simulink model "turbo_controller"  (R2025a)
settings: Solver=FixedStepAuto  StartTime=0.0  StopTime=inf  FixedStep=0.001  RelTol=1e-3
PostLoadFcn:
  | % 自动定位同目录CubeMX文件；不需要外部初始化脚本。
  | codertarget.data.setParameterValue('turbo_controller','STM32CubeMX.ProjectFile',fullfile(fileparts(get_param('turbo_controller','FileName')),'turbo_f407.ioc'));
InitFcn:
  | % 中文说明：按原控制器字段与类型创建三组接口总线；控制参数已内嵌。
  | tc_names=["EValve_Cycle" "EValve_Open" "Eblast_Cycle" "Eblast_Open" "Motor_Cycle" "Motor_Open" "EValve_Enable" "Eblast_Enable" "Motor_Enable" "SWO_Firework" "SWO_BleedAir" "EngineState" "Flag_ECUReset_Clear" "Flag_ECUReset_Save" "Flag_Reset_Enable" "Accelerator" "Nc_dem" "Nc"]; tc_types=["uint16" "uint16" "uint16" "uint16" "uint16" "uint16" "uint8" "uint8" "uint8" "uint8" "uint8" "uint8" "uint8" "uint8" "uint8" "single" "single" "single"];
  | for tc_k=1:numel(tc_names)
  |  tc_e(tc_k)=Simulink.BusElement; tc_e(tc_k).Name=char(tc_names(tc_k)); tc_e(tc_k).DataType=char(tc_types(tc_k));
  | end
  | EngineControl_Out=Simulink.Bus; EngineControl_Out.DataScope='Exported'; EngineControl_Out.Elements=tc_e;
  | clear tc_e tc_names tc_types tc_k
  | tc_names=["savedata1" "savedata2" "savedata3" "savedata4" "savedata5" "savedata6" "savedata7" "savedata8" "savedata9" "savedata10" "savedata11" "savedata12" "savedata13" "savedata14" "savedata15" "savedata16" "savedata17" "savedata18" "savedata19" "savedata20" "savedata21" "savedata22" "savedata23" "savedata24" "savedata25"]; tc_types=["single" "single" "single" "single" "single" "single" "single" "single" "single" "single" "single" "single" "single" "single" "single" "single" "single" "single" "single" "single" "single" "single" "single" "single" "single"];
  | for tc_k=1:numel(tc_names)
  |  tc_e(tc_k)=Simulink.BusElement; tc_e(tc_k).Name=char(tc_names(tc_k)); tc_e(tc_k).DataType=char(tc_types(tc_k));
  | end
  | SaveData_Out=Simulink.Bus; SaveData_Out.DataScope='Exported'; SaveData_Out.Elements=tc_e;
  | clear tc_e tc_names tc_types tc_k
  | tc_names=["senddata1" "senddata2" "senddata3" "senddata4" "senddata5" "senddata6" "senddata7" "senddata8" "senddata9" "senddata10" "senddata11" "senddata12" "senddata13" "senddata14" "senddata15" "senddata16" "senddata17" "senddata18" "senddata19" "senddata20" "senddata21" "senddata22" "senddata23" "senddata24" "senddata25" "senddata26" "senddata27" "senddata28" "senddata29"]; tc_types=["uint8" "uint8" "uint8" "uint8" "uint8" "uint8" "uint8" "uint8" "uint8" "uint8" "uint8" "uint8" "uint8" "uint8" "uint8" "uint8" "uint8" "uint8" "uint8" "uint8" "uint8" "uint8" "uint8" "uint8" "uint8" "uint8" "uint8" "uint8" "uint8"];
  | for tc_k=1:numel(tc_names)
  |  tc_e(tc_k)=Simulink.BusElement; tc_e(tc_k).Name=char(tc_names(tc_k)); tc_e(tc_k).DataType=char(tc_types(tc_k));
  | end
  | SendData_Out=Simulink.Bus; SendData_Out.DataScope='Exported'; SendData_Out.Elements=tc_e;
  | clear tc_e tc_names tc_types tc_k
  | 
  | % 以下为接口中文说明；只设置描述，不改变数值或数据类型。
  | EngineControl_Out.Description='执行控制输出（阀、电机、点火、状态及复位请求）';
  | tc_cn=["EValve_Cycle（主油阀周期计数（每计数2毫秒））" "EValve_Open（主油阀开通计数（每计数2毫秒））" "Eblast_Cycle（副油阀周期计数（每计数2毫秒））" "Eblast_Open（副油阀开通计数（每计数2毫秒））" "Motor_Cycle（起动电机周期计数）" "Motor_Open（起动电机开通计数）" "EValve_Enable（主油阀驱动使能）" "Eblast_Enable（副油阀驱动使能）" "Motor_Enable（起动电机使能）" "SWO_Firework（点火器使能（1开））" "SWO_BleedAir（引气阀使能（1开））" "EngineState（发动机状态）" "Flag_ECUReset_Clear（清除复位恢复状态请求）" "Flag_ECUReset_Save（保存复位恢复数据请求）" "Flag_Reset_Enable（处理器软件复位请求）" "Accelerator（油门／油泵给定控制量）" "Nc_dem（控制目标转速）" "Nc（发动机反馈转速（转每分））"];
  | tc_elements=EngineControl_Out.Elements;
  | for tc_k=1:numel(tc_cn)
  |  tc_elements(tc_k).Description=char(tc_cn(tc_k));
  | end
  | EngineControl_Out.Elements=tc_elements;
  | clear tc_cn tc_elements tc_k
  | SaveData_Out.Description='25项运行记录；字段含义按当前模型数据来源解释';
  | tc_cn=["savedata1（指令回显记录）" "savedata2（入口总温记录（℃））" "savedata3（电源电压记录）" "savedata4（排气温度记录（℃））" "savedata5（标定燃油压力记录）" "savedata6（副油阀占空比记录（％））" "savedata7（主油阀占空比记录（％））" "savedata8（温度修正转速记录）" "savedata9（开关输出及反馈位域）" "savedata10（物理转速记录）" "savedata11（油泵目标给定原始值）" "savedata12（起动电机占空比记录（％））" "savedata13（发动机状态码记录）" "savedata14（故障告警位域记录）" "savedata15（模型记录帧序号）" "savedata16（处理器温度记录（℃））" "savedata17（装订转速记录（沿用旧电源字段名））" "savedata18（导航高度记录）" "savedata19（飞行空速记录）" "savedata20（主阀旧记录位（恒零保留））" "savedata21（第21项保留记录（恒零））" "savedata22（保留记录项22）" "savedata23（保留记录项23）" "savedata24（保留记录项24）" "savedata25（保留记录项25）"];
  | tc_elements=SaveData_Out.Elements;
  | for tc_k=1:numel(tc_cn)
  |  tc_elements(tc_k).Description=char(tc_cn(tc_k));
  | end
  | SaveData_Out.Elements=tc_elements;
  | clear tc_cn tc_elements tc_k
  | SendData_Out.Description='29字段回传及外设命令接口；板端上位机帧只取第3至27字段';
  | tc_cn=["senddata1（回传发送允许标志（不直接上线路））" "senddata2（回传载荷长度25字节）" "senddata3（回传指令回显字节）" "senddata4（总温编码字节（℃＋80））" "senddata5（电源电压编码字节）" "senddata6（排温编码高字节）" "senddata7（排温编码低字节）" "senddata8（燃油压力编码高字节）" "senddata9（燃油压力编码低字节）" "senddata10（副油阀占空比字节（％））" "senddata11（主油阀占空比字节（％））" "senddata12（修正转速编码高字节）" "senddata13（修正转速编码低字节）" "senddata14（驱动及反馈状态位域）" "senddata15（物理转速编码高字节）" "senddata16（物理转速编码低字节）" "senddata17（油泵目标给定高字节（串口二使用））" "senddata18（油泵目标给定低字节（串口二使用））" "senddata19（起动电机占空比命令（串口一使用））" "senddata20（发动机状态码字节）" "senddata21（故障告警位域字节）" "senddata22（帧序号占位（板端另行填写））" "senddata23（处理器温度编码（℃＋50））" "senddata24（控制目标转速编码高字节）" "senddata25（控制目标转速编码低字节）" "senddata26（占位字节（板端改填实测泵速高字节））" "senddata27（占位字节（板端改填实测泵速低字节））" "senddata28（装订转速高字节（本板未发送））" "senddata29（装订转速低字节（本板未发送））"];
  | tc_elements=SendData_Out.Elements;
  | for tc_k=1:numel(tc_cn)
  |  tc_elements(tc_k).Description=char(tc_cn(tc_k));
  | end
  | SendData_Out.Elements=tc_elements;
  | clear tc_cn tc_elements tc_k
  | 
  | 
  | % FRAM模块化事务：接口类型和上电初始状态，随模型保存，无外部初始化文件。
  | clear FM_elements
  | FM_elements(1)=Simulink.BusElement;FM_elements(1).Name='phase';FM_elements(1).DataType='uint8';FM_elements(1).Dimensions=[1 1];FM_elements(1).Description='phase（当前事务阶段）';
  | FM_elements(2)=Simulink.BusElement;FM_elements(2).Name='a';FM_elements(2).DataType='uint8';FM_elements(2).Dimensions=[64 1];FM_elements(2).Description='a（启动时缓存的首区64字节）';
  | FM_elements(3)=Simulink.BusElement;FM_elements(3).Name='active';FM_elements(3).DataType='uint16';FM_elements(3).Dimensions=[1 1];FM_elements(3).Description='active（当前有效记录区地址）';
  | FM_elements(4)=Simulink.BusElement;FM_elements(4).Name='generation';FM_elements(4).DataType='uint32';FM_elements(4).Dimensions=[1 1];FM_elements(4).Description='generation（当前有效记录代号）';
  | FM_elements(5)=Simulink.BusElement;FM_elements(5).Name='record';FM_elements(5).DataType='uint8';FM_elements(5).Dimensions=[64 1];FM_elements(5).Description='record（本次冻结的待写记录）';
  | FM_elements(6)=Simulink.BusElement;FM_elements(6).Name='addr';FM_elements(6).DataType='uint16';FM_elements(6).Dimensions=[1 1];FM_elements(6).Description='addr（本次备用写入地址）';
  | FM_elements(7)=Simulink.BusElement;FM_elements(7).Name='lastSave';FM_elements(7).DataType='single';FM_elements(7).Dimensions=[1 1];FM_elements(7).Description='lastSave（上次开始保存的秒数）';
  | FM_elements(8)=Simulink.BusElement;FM_elements(8).Name='lastState';FM_elements(8).DataType='uint8';FM_elements(8).Dimensions=[1 1];FM_elements(8).Description='lastState（上次保存时的发动机状态）';
  | FM_elements(9)=Simulink.BusElement;FM_elements(9).Name='boot';FM_elements(9).DataType='boolean';FM_elements(9).Dimensions=[1 1];FM_elements(9).Description='boot（启动记录是否允许恢复）';
  | FM_elements(10)=Simulink.BusElement;FM_elements(10).Name='consumed';FM_elements(10).DataType='boolean';FM_elements(10).Dimensions=[1 1];FM_elements(10).Description='consumed（本次启动恢复通知是否已发送）';
  | FM_elements(11)=Simulink.BusElement;FM_elements(11).Name='payload';FM_elements(11).DataType='uint8';FM_elements(11).Dimensions=[20 1];FM_elements(11).Description='payload（当前20字节恢复内容）';
  | ... (+35 lines)
model workspace (MAT data in the model file):
  CRC16_Table_Reference = [0 4129 8258 12387 16516 20645 24774 28903 33032 37161 41290 45419 ... (256 elements, 256x1)]
  PE_Kaer = [0.15402 0.15402 0.12264 0.10076 0.09481 0.07601 0.07111 0.0569 0.05198 0.04926 0.05308 0.04325 ... (13 elements, 1x13)]
  PE_Nr = [21.2982 61.4260372 67.7475458 72.7394382 76.845934 80.6988798 83.8449282 86.6491912 88.9382406 89.178606 91.1938214 93.4068058 ... (13 elements, 1x13)]
  PE_Pump_Translate = 33.5999984741
  PE_RotaSpeed_Translate = 860
  PE_Taer = [0.4939154 0.4939154 0.40780982 0.34066978 0.31622756 0.30405716 0.34300244 0.26785022 0.37393554 0.23914836 0.44563948 0.31044662 ... (13 elements, 1x13)]
  PF_ACCFULLRANGE = 3360
  PF_Flag_ECUReset = 0
  PF_Flag_rx_suc = 1
  PF_Gear_Info = [40000; 45000; 50000; 55000; 57000; 59000; 60000; 61000; 61000; 61000; 61000; 61000]
  PF_K_TiaoJie = 1
  PF_Kpu = 10
  PF_MySet_Rxdata = [0 0 0 0 0 0 0 0 0 0 0 0 ... (50 elements, 50x1)]
  PF_MyUsart1_Rxdata = [0 0 0 0 0 0 0 0 0 0 0 0 ... (50 elements, 50x1)]
  PF_MyUsart2_Rxdata = [0 0 0 0 0 0 0 0 0 0 0 0 ... (50 elements, 50x1)]
  PF_Reset_Information = [0 0 0 0 0 0 0 0 0 0 0 0 ... (20 elements, 20x1)]
  PF_Sensor_X1_T4 = [0 4095]
  PF_Sensor_X2_T4 = [0 1.66666698456]
  PF_Sensor_X3_T4 = [0 504 999 1497 2010 2529 3051 3568 4076 4571 4959]
  PF_Sensor_X_P2 = [0.5 3]
  PF_Sensor_X_Poil = [0.5 3]
  PF_Sensor_X_T1t = [-50 300]
  PF_Sensor_X_Vpower = [0 3]
  PF_Sensor_X_Vpump = [0 3]
  PF_Sensor_Y1_T4 = [0 3]
  PF_Sensor_Y2_T4 = [0 5000]
  PF_Sensor_Y3_T4 = [0 100 200 300 400 500 600 700 800 900 980]
  PF_Sensor_Y_P2 = [0 1000]
  PF_Sensor_Y_Poil = [0 1000]
  PF_Sensor_Y_T1t = [-50 300]
  PF_Sensor_Y_Vpower = [0 33]
  PF_Sensor_Y_Vpump = [0 33]
  PG_CtrlMode_CloseLoop : mpt.Parameter (value not decoded)
  PG_CtrlMode_ManualAcc : mpt.Parameter (value not decoded)
  PG_CtrlMode_Origin : mpt.Parameter (value not decoded)
  PG_CtrlMode_Start : mpt.Parameter (value not decoded)
  PG_CtrlMode_Stop : mpt.Parameter (value not decoded)
  PG_ES_Clp : mpt.Parameter (value not decoded)
  PG_ES_EngStart : mpt.Parameter (value not decoded)
  PG_ES_Manual : mpt.Parameter (value not decoded)
  PG_ES_Origin : mpt.Parameter (value not decoded)
  PG_ES_Stop : mpt.Parameter (value not decoded)
  PG_Instr_BleedAirSet : mpt.Parameter (value not decoded)
  PG_Instr_CloseLoop : mpt.Parameter (value not decoded)
  PG_Instr_ECUReSet : mpt.Parameter (value not decoded)
  PG_Instr_EValveSet : mpt.Parameter (value not decoded)
  PG_Instr_EblastSet : mpt.Parameter (value not decoded)
  PG_Instr_Erase : mpt.Parameter (value not decoded)
  PG_Instr_FireWorkSet : mpt.Parameter (value not decoded)
  PG_Instr_ManualPlus : mpt.Parameter (value not decoded)
  PG_Instr_ManualrReduce : mpt.Parameter (value not decoded)
  PG_Instr_MotorSet : mpt.Parameter (value not decoded)
  PG_Instr_OilSet : mpt.Parameter (value not decoded)
  PG_Instr_SelfCheck : mpt.Parameter (value not decoded)
  PG_Instr_Start : mpt.Parameter (value not decoded)
  PG_Instr_Stop : mpt.Parameter (value not decoded)
  PG_Instr_StopZero : Simulink.Parameter (value not decoded)
  PG_Location_Air : Simulink.Parameter (value not decoded)
  PG_Location_Gnd : Simulink.Parameter (value not decoded)
  PG_ServoCtrlMode_CloseLoop : Simulink.Parameter (value not decoded)
  PG_ServoCtrlMode_CloseLoopMax : Simulink.Parameter (value not decoded)
  PG_ServoCtrlMode_CloseLoopMin : Simulink.Parameter (value not decoded)
  PG_ServoCtrlMode_ManualAcc : Simulink.Parameter (value not decoded)
  PG_ServoCtrlMode_ManualAccMax : Simulink.Parameter (value not decoded)
  PG_ServoCtrlMode_ManualAccMin : Simulink.Parameter (value not decoded)
  PG_SpeedDot_Permit : Simulink.Parameter (value not decoded)
  PL_EngineModel_Actuator = [0 10 100]
  PL_EngineModel_EngineStar_Press_P2 = [1013 1098.4 1099.144828 1099.931034 1103.613793 1162.662069 1143.793103 1131.006897 1123.186207 1117.6 1114 1111.806897 ... (127 elements, 1x127)]
  PL_EngineModel_EngineStar_RotaSpeed = [200 2000 9584 9660 10220 10240 10260 10288 10308 10368 10380 10408 ... (127 elements, 1x127)]
  PL_EngineModel_EngineStar_Temp_Exhaust = [128 129 129.1 130 131 131.1 132 133 134 134.1 135 135.1 ... (127 elements, 1x127)]
  PL_EngineModel_EngineStar_Time = [0.05 0.1 0.15 0.2 0.25 0.3 0.35 0.4 0.45 0.5 0.55 0.6 ... (127 elements, 1x127)]
  PL_EngineModel_IdleAbove_Nr = [0 21.2982 61.4260372 67.7475458 72.7394382 76.845934 80.6988798 83.8449282 86.6491912 88.9382406 89.178606 91.1938214 ... (14 elements, 1x14)]
  PL_EngineModel_IdleAbove_P2r = [0.986923266716 1.57907722675 1.81593881076 1.99358499877 2.23044658278 2.43770046879 2.65482358747 2.84233900814 3.03972366149 3.18776215149 3.25684678016 3.3950160375 ... (14 elements, 1x14)]
  PL_EngineModel_IdleAbove_Tempr = [0.0536001429337 1.07200285867 1.63301768805 1.63659103091 1.66875111667 1.72592460247 1.77595140254 1.86171163123 1.95461854565 2.03323208862 2.03323208862 2.13685903162 ... (14 elements, 1x14)]
  PL_EngineModel_IdleAbove_Ter = [0.42434128 0.42434128 0.42434128 0.30669408 0.23570008 0.22150128 0.1997974 0.23803274 0.16115638 0.24279948 0.13600422 0.31308354 ... (14 elements, 1x14)]
  PL_EngineModel_IdleAbove_Wfr = [0 10.142 23.8337 27.8905 31.9473 36.0041 40.0609 44.1177 48.1745 52.2313 52.7384 56.7952 ... (14 elements, 1x14)]
  PL_EngineModel_Press_P2 = [400 400 400 400 400 400 400 400 400 400]
  PL_EngineModel_Rotaspeed = [0 20000 96400]
  PL_EngineModel_Temp_Exhaust = [500 500 500 500 500 500 500 500 500 500]
  PL_Kaer = [0.1 0.1 0.1 0.1 0.1 0.1]
  PL_Nr = [50 60 70 80 90 100]
  PL_Taer = [0.1 0.1 0.1 0.1 0.1 0.1]
  Sig : Simulink.Signal (value not decoded)
  Ts_ms : Simulink.Parameter (value not decoded)
  false : Simulink.Parameter (value not decoded)
  true : Simulink.Parameter (value not decoded)
symbols that are objects in the model workspace (value not decoded): PG_CtrlMode_CloseLoop, PG_CtrlMode_ManualAcc, PG_CtrlMode_Origin, PG_CtrlMode_Start, PG_CtrlMode_Stop, PG_ES_Clp, PG_ES_EngStart, PG_ES_Manual, PG_ES_Origin, PG_ES_Stop, PG_Instr_BleedAirSet, PG_Instr_CloseLoop, PG_Instr_EblastSet, PG_Instr_ECUReSet, PG_Instr_Erase, PG_Instr_EValveSet, PG_Instr_FireWorkSet, PG_Instr_ManualPlus, PG_Instr_ManualrReduce, PG_Instr_MotorSet, PG_Instr_OilSet, PG_Instr_SelfCheck, PG_Instr_Start, PG_Instr_Stop, PG_Instr_StopZero, PG_ServoCtrlMode_CloseLoop, PG_ServoCtrlMode_CloseLoopMax, PG_ServoCtrlMode_CloseLoopMin, PG_ServoCtrlMode_ManualAcc, PG_ServoCtrlMode_ManualAccMax, PG_ServoCtrlMode_ManualAccMin, Ts_ms
libraries: simulink x97, stm32blockslib x10, stm32f4xxblockslib x8
(part 5 of 26)

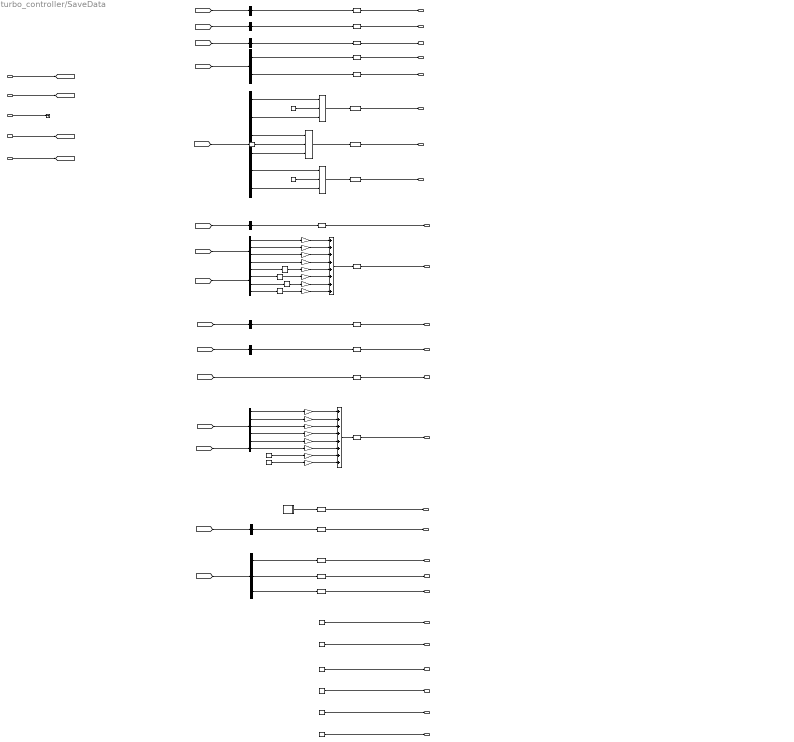
== system turbo_controller/SaveData ==
  note: SaveData的职责：整理25项运行记录，不直接写文件
      |
      | 从发动机模式、传感器/通信、执行输出和监视告警中取出需要记录的量，按固定25个输出端口排列，
      | 供后面的Savedata总线和LogPack使用。
      |
      | 多数通道只转换为single，不额外加偏置、不拆高低字节。阀门和电机另计算开通比例；开关和告警另
      | 组合为位字段；Hold另产生循环序号。
      |
      | S_ClM_Parameter输入当前直接接Terminator，未参与这些记录。第20～25项目前全部是固定0，不应沿
      | 用旧名称推断这些项已经存了主阀输出、软件版本或其他传感器量。
      |
      | 本页没有文件路径、SD卡写入、SPI写入或串口封帧动作。它提供一组记录字段；实际数据去向还要继
      | 续看LogPack、SDLog和FRAM事务。
  note: 温度、电压、油压和转速：保留数值，不按回传字节编码
      |
      | 第2项T0取Sensor.T0，直接转single，25 ℃仍记录25，不加80。
      | 第3项dianyuandianya取Sensor.Vpower，24 V仍记录24，不乘5。
      | 第4项T4取Sensor.T4_Filter，第5项POil取Sensor.POil_Filter，保留滤波后的值，不拆成两个字节；
      | 油压单位沿用上游标定。
      | 第8项HuanSuanZhuanSu取温度修正转速，第10项WuLiZhuanSu取Sensor.Origin_Nc，保留完整转速，不
      | 除2。
      | 第16项Tecu取Sensor.Tecu，25 ℃仍记录25，不加50。
      | 第11项NBump_MuBiao取执行输出Accelerator，是泵控制给定编码，不是实测泵速。
      |
      | 这些转换的输出类型是single。即使参数页上写有Floor，也不能据此说这里全部取整；浮点转single
      | 不等于转整数，原有小数一般仍保留到single精度。
  note: 阀门和电机记录的是开通比例，不是机械反馈
      |
      | 从S_Servo_Out取Open及Cycle，计算：
      | 第6项副油阀=100×Eblast_Open/Eblast_Cycle；
      | 第7项主油阀=100×EValve_Open/EValve_Cycle；
      | 第12项电机=100×Motor_Open/Motor_Cycle。
      | 结果转single记录，此处没有再转成uint8或强制向下取整。
      |
      | 例周期30、开通15，记录50，代表50%开通比例；周期30、开通10，约为33.3333。它不是开了15 ms，
      | 也不是阀芯走到50%的位置。
      |
      | 这些量来自驱动设定，使能状态另在第9项位字段里。比例非0不自动证明执行器已经动作。本页沿用原
      | 除法，没有在这里增加分母为0时的保护逻辑；本次仅更新说明。
  note: 第9项开关量：命令和取反反馈合成一个数
      |
      | 低四位来自执行输出，高四位来自传感器反馈的逻辑取反：
      | 位0，权重1：SWO_Firework点火使能；
      | 位1，权重2：EValve_Enable主阀使能；
      | 位2，权重4：Eblast_Enable副阀使能；
      | 位3，权重8：SWO_BleedAir引气使能；
      | 位4，权重16：NOT SWI_Firework；
      | 位5，权重32：NOT SWI_EValve；
      | 位6，权重64：NOT SWI_Eblast；
      | 位7，权重128：NOT SWI_BleedAir。
      |
      | 按各位权重相加后转single存储。例只有主阀使能和取反后的主阀反馈为真，记录2+32=34。分析日志
      | 时先转成整数再按位拆解，不要把34当成开度34%。
      |
      | Motor_Enable没有放入这8位；电机开通比例在第12项。高四位与原反馈相反，不能直接当作GPIO原电
      | 平解释。
  note: 第14项告警字段：与SendData的定义存在差别
      |
      | 各布尔量乘位权后相加，结果转single：
      | 位0（1）：Alarm_OverTemp；
      | 位1（2）：Alarm_OverSpeed；
      | 位2（4）：Flag_NcFailure；
      | 位3（8）：Alarm_ECUReset；
      | 位4（16）：Alarm_Vpower_Low；
      | 位5（32）：Sensor.SWI_ValveErr原值；
      | 位6（64）：当前常量0；
      | 位7（128）：当前常量0。
      |
      | 例如超温、欠压为真，其余为假，得到17。这里的位5直接使用SWI_ValveErr，没有NOT；SendData对应
      | 位使用了NOT，不能拿同一套解码说明混用。这里的位6也没有接Lock_NcFailure，记录0不表示该锁存
      | 故障一定不存在。
      |
      | 本页只组合并记录标志，不触发报警、停车或复位。判断运行状态要另外看第13项模式编号。
  note: 25项顺序表：第1～13项
      |
      | 1 ZhiLingHuiChuan：COMM.Instr_XianShi，指令回显。
      | 2 T0：入口温度，直接single。
      | 3 dianyuandianya：Sensor.Vpower，供电电压原值。
      | 4 T4：滤波后排温。
      | 5 POil：滤波后油压。
      | 6 Eblast：副油阀开通比例，100×Open/Cycle。
      | 7 EValve：主油阀开通比例，100×Open/Cycle。
      | 8 HuanSuanZhuanSu：温度修正转速完整值。
      | 9 KaiGuanLiang：命令与取反反馈的8位组合。
      | 10 WuLiZhuanSu：Sensor.Origin_Nc完整值。
      | 11 NBump_MuBiao：Accelerator泵给定控制编码。
      | 12 Motor：电机开通比例，100×Open/Cycle。
      | 13 FaDongJiZhuangTai：EngineState，0初始、1普通起动、2闭环、3手动、4停车。
      |
      | 这些是记录项/输出端口编号，不是串口帧字节位置。第13项是发动机模式，不是指令编号或起动A～F
      | 阶段。
  note: 25项顺序表：第14～25项及旧名称说明
      |
      | 14 GuZhangXingXi：告警位组合，按本页专用位定义解码。
      | 15 zhenjishu：Hold产生的0～255循环序号。
      | 16 Tecu：Sensor.Tecu处理器温度原值，不加50。
      | 17 DianYuan：实际为COMM.SpeedLoad目标/装订转速，不是电源电压。
      | 18 H：COMM.H_Gprs导航高度，沿用输入单位，本页不作单位换算。
      | 19 speed：COMM.AirSpeed飞行空速；不是发动机轴转速。
      | 20 ZhuFaShuChu：当前固定0，不是有效主阀反馈。
      | 21 名称为12：当前固定0，此名字不表示第12项。
      | 22 BeiYong1：固定0。
      | 23 BeiYong2：固定0。
      | 24 BeiYong3：固定0。
      | 25 BeiYong4：固定0。
      |
      | 第17项还会以savedata17被FRAM打包步骤读取，作为恢复记录中的目标转速。若把它误认为电压，会连
      | 带误读恢复信息。真正供电在第3项。
  note: Hold序号与最终27项日志的关系
      |
      | Hold每次执行时判断Out是否达到255：达到则置0，否则加1。序列循环为…253、254、255、0、1…；
      | 第15项把这个序号转single记录。
      |
      | 它是本图执行次数的循环标记，不是时间戳。重复的序号不一定表示重复数据，因为每256次执行就回
      | 到同一编号；不要把序号差直接解释成秒数。
      |
      | 外层LogPack按savedata1～savedata25拼接本页25项，末尾追加第26项时间（秒）和第27项FRAM写后验
      | 证失败次数，形成27×1的single向量。随后SDLog的To Workspace在仿真中生成engine_log。
      |
      | 这里的27项是数值记录，不是27字节帧；名为SDLog也不能单凭名称断言已写入实际SD卡。实际记录周
      | 期取决于外层执行与记录接口，本页没有独立的周期触发器。
  note: 读日志时不要套用SendData的还原规则
      |
      | SaveData与SendData虽然记录同类变量，表示方式不同：
      | 日志T0直接是温度；回传T0加80。
      | 日志Tecu直接是温度；回传Tecu加50且限幅。
      | 日志电压直接是V；回传电压乘5。
      | 日志转速保留完整值；回传部分转速除2并拆字节。
      | 日志主副阀、电机比例是single，可有小数；回传比例转uint8。
      | 日志告警位5是SWI_ValveErr原值，位6为0；回传位5取反，位6接Lock_NcFailure。
      |
      | 例如日志中T0=25、电压=24、转速=50000，应按这些数直接阅读，不能再减80、除5或乘2。开关与告警
      | 则需要按位解析，泵给定仍是控制编码。所有项统一转single不意味着所有项拥有相同单位。
  S_EngineState : Inport
      settings: AttributesFormatString=S_EngineState（发动机状态）
  S_SPM : Inport  Port=2
      settings: AttributesFormatString=S_SPM（通信及传感器信息总线）
  S_ClM_Parameter : Inport  Port=3
      settings: AttributesFormatString=S_ClM_Parameter（控制规律管理模块参数）
  S_Servo_Out : Inport  Port=4
      settings: AttributesFormatString=S_Servo_Out（伺服输出）
  S_MAlarm : Inport  Port=5
      settings: AttributesFormatString=S_MAlarm（报警）
  Bus Selector1 : BusSelector  OutputSignals=Sensor（传感器信息总线）.T0（入口总温）
      settings: AttributesFormatString=Bus Selector1（总线选择器1）
  Bus Selector10 : BusSelector  OutputSignals=EValve_Open（主油阀开通计数）,EValve_Cycle（主油阀周期计数）,Eblast_Open（副油阀开通计数）,Eblast_Cycle（副油阀周期计数）,Motor_Open（起动电机开通计数）,Motor_Cycle（起动电机周期计数）
      settings: AttributesFormatString=Bus Selector10（总线选择器10）
  Bus Selector11 : BusSelector  OutputSignals=SWO_Firework（点火器使能）,EValve_Enable（主油阀使能）,Eblast_Enable（副油阀使能）,SWO_BleedAir（引气阀使能）
      settings: AttributesFormatString=Bus Selector11（总线选择器11）
  Bus Selector12 : BusSelector  OutputSignals=Sensor（传感器信息总线）.Tecu（处理器温度）
      settings: AttributesFormatString=Bus Selector12（总线选择器12）
  Bus Selector13 : BusSelector  OutputSignals=COMM（通信信息总线）.Instr_XianShi（指令回显）
      settings: AttributesFormatString=Bus Selector13（总线选择器13）
  Bus Selector14 : BusSelector  OutputSignals=Sensor（传感器信息总线）.SWI_Firework（点火器告警反馈）,Sensor（传感器信息总线）.SWI_EValve（主油阀反馈）,Sensor（传感器信息总线）.SWI_Eblast（副油阀反馈）,Sensor（传感器信息总线）.SWI_BleedAir（引气阀反馈）
      settings: AttributesFormatString=Bus Selector14（总线选择器14）
  Bus Selector15 : BusSelector  OutputSignals=Accelerator（油泵给定控制量）
      settings: AttributesFormatString=Bus Selector15（总线选择器15）
  Bus Selector17 : BusSelector  OutputSignals=Sensor（传感器信息总线）.HuanSuanZhuanSu（温度修正转速）
      settings: AttributesFormatString=Bus Selector17（总线选择器17）
  Bus Selector18 : BusSelector  OutputSignals=Sensor（传感器信息总线）.SWI_ValveErr（阀门综合告警反馈）
      settings: AttributesFormatString=Bus Selector18（总线选择器18）
  Bus Selector2 : BusSelector  OutputSignals=Sensor（传感器信息总线）.T4_Filter（滤波后排气温度）,Sensor（传感器信息总线）.POil_Filter（滤波后燃油压力）
      settings: AttributesFormatString=Bus Selector2（总线选择器2）
  Bus Selector3 : BusSelector  OutputSignals=Sensor（传感器信息总线）.Vpower（电源电压）
      settings: AttributesFormatString=Bus Selector3（总线选择器3）
  Bus Selector4 : BusSelector  OutputSignals=Sensor（传感器信息总线）.Origin_Nc（原位转速）
      settings: AttributesFormatString=Bus Selector4（总线选择器4）
  Bus Selector8 : BusSelector  OutputSignals=COMM（通信信息总线）.SpeedLoad（装订转速）,COMM（通信信息总线）.H_Gprs（导航高度）,COMM（通信信息总线）.AirSpeed（飞行空速）
      settings: AttributesFormatString=Bus Selector8（总线选择器8）
  Bus Selector9 : BusSelector  OutputSignals=Alarm_OverTemp（超温告警）,Alarm_OverSpeed（超转告警）,Flag_NcFailure（转速传感器故障标志）,Alarm_ECUReset（控制器复位告警）,Alarm_Vpower_Low（电源欠压告警）
      settings: AttributesFormatString=Bus Selector9（总线选择器9）
  Data Type Conversion{1..9,11..16,19..20,22,24} (19 alike) : DataTypeConversion  OutDataTypeStr=single  SaturateOnIntegerOverflow=off  RndMeth=Floor
      Data Type Conversion1 settings: AttributesFormatString=Data Type Conversion1（数据类型转换1）
      Data Type Conversion11 settings: AttributesFormatString=Data Type Conversion11（数据类型转换11）
      Data Type Conversion12 settings: AttributesFormatString=Data Type Conversion12（数据类型转换12）
      Data Type Conversion13 settings: AttributesFormatString=Data Type Conversion13（数据类型转换13）
      Data Type Conversion14 settings: AttributesFormatString=Data Type Conversion14（数据类型转换14）
      Data Type Conversion15 settings: AttributesFormatString=Data Type Conversion15（数据类型转换15）
      Data Type Conversion16 settings: AttributesFormatString=Data Type Conversion16（数据类型转换16）
      Data Type Conversion19 settings: AttributesFormatString=Data Type Conversion19（数据类型转换19）
      Data Type Conversion2 settings: AttributesFormatString=Data Type Conversion2（数据类型转换2）
      Data Type Conversion20 settings: AttributesFormatString=Data Type Conversion20（数据类型转换20）
      Data Type Conversion22 settings: AttributesFormatString=Data Type Conversion22（数据类型转换22）
      Data Type Conversion24 settings: AttributesFormatString=Data Type Conversion24（数据类型转换24）
      Data Type Conversion3 settings: AttributesFormatString=Data Type Conversion3（数据类型转换3）
      Data Type Conversion4 settings: AttributesFormatString=Data Type Conversion4（数据类型转换4）
      Data Type Conversion5 settings: AttributesFormatString=Data Type Conversion5（数据类型转换5）
      Data Type Conversion6 settings: AttributesFormatString=Data Type Conversion6（数据类型转换6）
      Data Type Conversion7 settings: AttributesFormatString=Data Type Conversion7（数据类型转换7）
      Data Type Conversion8 settings: AttributesFormatString=Data Type Conversion8（数据类型转换8）
      Data Type Conversion9 settings: AttributesFormatString=Data Type Conversion9（数据类型转换9）
  Gain1 : Gain  OutDataTypeStr=uint8
      settings: AttributesFormatString=Gain1（乘以系数1）
  Gain10 : Gain  Gain=16  OutDataTypeStr=uint8
      settings: AttributesFormatString=Gain10（乘以系数16）
  Gain11 : Gain  Gain=32  OutDataTypeStr=uint8
      settings: AttributesFormatString=Gain11（乘以系数32）
  Gain12 : Gain  Gain=64  OutDataTypeStr=uint8
      settings: AttributesFormatString=Gain12（乘以系数64）
  Gain13 : Gain  Gain=128  OutDataTypeStr=uint8
      settings: AttributesFormatString=Gain13（乘以系数128）
  Gain14 : Gain  Gain=2  OutDataTypeStr=uint8
      settings: AttributesFormatString=Gain14（乘以系数2）
  Gain15 : Gain  Gain=4  OutDataTypeStr=uint8
      settings: AttributesFormatString=Gain15（乘以系数4）
  Gain16 : Gain  Gain=8  OutDataTypeStr=uint8
      settings: AttributesFormatString=Gain16（乘以系数8）
  Gain2 : Gain  Gain=16  OutDataTypeStr=uint8
      settings: AttributesFormatString=Gain2（乘以系数16）
  Gain3 : Gain  Gain=32  OutDataTypeStr=uint8
      settings: AttributesFormatString=Gain3（乘以系数32）
  Gain4 : Gain  Gain=64  OutDataTypeStr=uint8
      settings: AttributesFormatString=Gain4（乘以系数64）
  Gain5 : Gain  Gain=128  OutDataTypeStr=uint8
      settings: AttributesFormatString=Gain5（乘以系数128）
  Gain6 : Gain  Gain=2  OutDataTypeStr=uint8
      settings: AttributesFormatString=Gain6（乘以系数2）
  Gain7 : Gain  Gain=4  OutDataTypeStr=uint8
      settings: AttributesFormatString=Gain7（乘以系数4）
  Gain8 : Gain  Gain=8  OutDataTypeStr=uint8
      settings: AttributesFormatString=Gain8（乘以系数8）
  Gain9 : Gain  OutDataTypeStr=uint8
      settings: AttributesFormatString=Gain9（乘以系数1）
  Hold : Stateflow chart  Description=|  TreatAsAtomicUnit=on  RTWFcnName=Timmer  RTWFileName=EngineControl_Timmer
      | 产生0～255循环的记录序号
      | 
      | 每次执行先判断当前Out是否已达到255：达到就置0，否则加1。序列循环为…253、254、255、0、1…。
      | 
      | 这里先判断再递增，避免uint8在255上继续加1触发溢出诊断。它是记录顺序标记，不是秒数；记录间隔取决于父级调用频率。一个序号重复出现也不一定表示数据重复，因为每256次调用会正常回到相同编号。
      settings: AttributesFormatString=Hold（保持）  RTWSystemCode=Reusable function  RTWFcnNameOpts=Use subsystem name  RTWFileNameOpts=User specified
  Logical Operator{,1..3} (4 alike) : Logic  Operator=NOT  AllPortsSameDT=off  OutDataTypeStr=boolean
      Logical Operator settings: AttributesFormatString=Logical Operator（逻辑运算）
      Logical Operator1 settings: AttributesFormatString=Logical Operator1（逻辑运算1）
      Logical Operator2 settings: AttributesFormatString=Logical Operator2（逻辑运算2）
      Logical Operator3 settings: AttributesFormatString=Logical Operator3（逻辑运算3）
  Product1 : Product  Inputs=**/
      settings: AttributesFormatString=Product1（乘法1）
  Product3 : Product  Inputs=**/
      settings: AttributesFormatString=Product3（乘法3）
  Product7 : Product  Inputs=**/
      settings: AttributesFormatString=Product7（乘法7）
  Sum of Elements1 : Sum  Inputs=++++++++
      settings: AttributesFormatString=Sum of Elements1（加法求和的元素1）
  Sum of Elements4 : Sum  Inputs=++++++++
      settings: AttributesFormatString=Sum of Elements4（加法求和的元素4）
  Terminator : Terminator
      settings: AttributesFormatString=Terminator（终止未使用信号）
  dth = T0-288.1 : Constant  Value=100  OutDataTypeStr=single  SampleTime=-1
      settings: AttributesFormatString=dth = T0-288.1（固定常量100（旧名称不参与计算））
  dth = T0-288.{2,4..8,10..11} (8 alike) : Constant  Value=0  OutDataTypeStr=single  SampleTime=-1
      dth = T0-288.10 settings: AttributesFormatString=dth = T0-288.10（固定常量0（旧名称不参与计算））
      dth = T0-288.11 settings: AttributesFormatString=dth = T0-288.11（固定常量0（旧名称不参与计算））
      dth = T0-288.2 settings: AttributesFormatString=dth = T0-288.2（固定常量0（旧名称不参与计算））
      dth = T0-288.4 settings: AttributesFormatString=dth = T0-288.4（固定常量0（旧名称不参与计算））
      dth = T0-288.5 settings: AttributesFormatString=dth = T0-288.5（固定常量0（旧名称不参与计算））
      dth = T0-288.6 settings: AttributesFormatString=dth = T0-288.6（固定常量0（旧名称不参与计算））
      dth = T0-288.7 settings: AttributesFormatString=dth = T0-288.7（固定常量0（旧名称不参与计算））
      dth = T0-288.8 settings: AttributesFormatString=dth = T0-288.8（固定常量0（旧名称不参与计算））
  dth = T0-288.13 : Constant  Value=100  OutDataTypeStr=single  SampleTime=-1
      settings: AttributesFormatString=dth = T0-288.13（固定常量100（旧名称不参与计算））
  dth = T0-288.9 : Constant  Value=100  OutDataTypeStr=single  SampleTime=-1
      settings: AttributesFormatString=dth = T0-288.9（固定常量100（旧名称不参与计算））
  ZhiLingHuiChuan : Outport  Description=记录项1 ZhiLingHuiChuan：指令回显COMM.Instr_XianShi。作为savedata1进入固定日志顺序，不是字节编号。
      settings: AttributesFormatString=ZhiLingHuiChuan（指令回显记录）
  T0 : Outport  Description=记录项2 T0：入口温度T0原值，single，不加80。作为savedata2进入固定日志顺序，不是字节编号。  Port=2
      settings: AttributesFormatString=T0（入口总温记录（℃））
  dianyuandianya : Outport  Description=记录项3 dianyuandianya：供电电压Vpower原值，single，不乘5。作为savedata3进入固定日志顺序，不是字节编号。  Port=3
      settings: AttributesFormatString=dianyuandianya（电源电压记录）
  T4 : Outport  Description=记录项4 T4：T4_Filter滤波排温原值。作为savedata4进入固定日志顺序，不是字节编号。  Port=4
      settings: AttributesFormatString=T4（排气温度记录（℃））
  POil : Outport  Description=记录项5 POil：POil_Filter滤波油压原值。作为savedata5进入固定日志顺序，不是字节编号。  Port=5
      settings: AttributesFormatString=POil（标定燃油压力记录）
  Eblast : Outport  Description=记录项6 Eblast：副油阀100×Open/Cycle，single比例。作为savedata6进入固定日志顺序，不是字节编号。  Port=6
      settings: AttributesFormatString=Eblast（副油阀占空比记录（％））
  EValve : Outport  Description=记录项7 EValve：主油阀100×Open/Cycle，single比例。作为savedata7进入固定日志顺序，不是字节编号。  Port=7
      settings: AttributesFormatString=EValve（主油阀占空比记录（％））
  HuanSuanZhuanSu : Outport  Description=记录项8 HuanSuanZhuanSu：温度修正转速完整值，不除2。作为savedata8进入固定日志顺序，不是字节编号。  Port=8
      settings: AttributesFormatString=HuanSuanZhuanSu（温度修正转速记录）
  KaiGuanLiang : Outport  Description=记录项9 KaiGuanLiang：命令与取反反馈的8位组合。作为savedata9进入固定日志顺序，不是字节编号。  Port=9
      settings: AttributesFormatString=KaiGuanLiang（开关输出及反馈位域）
  WuLiZhuanSu : Outport  Description=记录项10 WuLiZhuanSu：Origin_Nc完整转速，不除2。作为savedata10进入固定日志顺序，不是字节编号。  Port=10
      settings: AttributesFormatString=WuLiZhuanSu（物理转速记录）
  NBump_MuBiao : Outport  Description=记录项11 NBump_MuBiao：Accelerator泵给定控制编码，不是实测泵速。作为savedata11进入固定日志顺序，不是字节编号。  Port=11
      settings: AttributesFormatString=NBump_MuBiao（油泵目标给定原始值）
  Motor : Outport  Description=记录项12 Motor：电机100×Open/Cycle，single比例。作为savedata12进入固定日志顺序，不是字节编号。  Port=12
      settings: AttributesFormatString=Motor（起动电机占空比记录（％））
  FaDongJiZhuangTai : Outport  Description=记录项13 FaDongJiZhuangTai：发动机模式0初始1普通起动2闭环3手动4停车。作为savedata13进入固定日志顺序，不是字节编号。  Port=13
      settings: AttributesFormatString=FaDongJiZhuangTai（发动机状态码记录）
  GuZhangXingXi : Outport  Description=记录项14 GuZhangXingXi：告警位组合；位5为SWI_ValveErr原值，位6/7固定0。作为savedata14进入固定日志顺序，不是字节编号。  Port=14
      settings: AttributesFormatString=GuZhangXingXi（故障告警位域记录）
  zhenjishu : Outport  Description=记录项15 zhenjishu：0～255循环记录序号，不是秒数。作为savedata15进入固定日志顺序，不是字节编号。  Port=15
      settings: AttributesFormatString=zhenjishu（模型记录帧序号）
  Tecu : Outport  Description=记录项16 Tecu：处理器温度Tecu原值，不加50。作为savedata16进入固定日志顺序，不是字节编号。  Port=16
      settings: AttributesFormatString=Tecu（处理器温度记录（℃））
  DianYuan : Outport  Description=记录项17 DianYuan：COMM.SpeedLoad目标转速；旧名DianYuan不表示电压。作为savedata17进入固定日志顺序，不是字节编号。  Port=17
      settings: AttributesFormatString=DianYuan（装订转速记录（沿用旧电源字段名））
  H : Outport  Description=记录项18 H：COMM.H_Gprs导航高度；本页不换算单位。作为savedata18进入固定日志顺序，不是字节编号。  Port=18
      settings: AttributesFormatString=H（导航高度记录）
  speed : Outport  Description=记录项19 speed：COMM.AirSpeed飞行空速，不是发动机转速。作为savedata19进入固定日志顺序，不是字节编号。  Port=19
      settings: AttributesFormatString=speed（飞行空速记录）
  ZhuFaShuChu : Outport  Description=记录项20 ZhuFaShuChu：固定0；旧名不表示已有主阀反馈。作为savedata20进入固定日志顺序，不是字节编号。  Port=20
      settings: AttributesFormatString=ZhuFaShuChu（主阀旧记录位（恒零保留））
  12 : Outport  Description=记录项21 12：固定0；端口旧名12不表示第12项。作为savedata21进入固定日志顺序，不是字节编号。  Port=21
      settings: AttributesFormatString=12（第21项保留记录（恒零））
  BeiYong1 : Outport  Description=记录项22 BeiYong1：备用常量0。作为savedata22进入固定日志顺序，不是字节编号。  Port=22
      settings: AttributesFormatString=BeiYong1（保留记录项22）
  BeiYong2 : Outport  Description=记录项23 BeiYong2：备用常量0。作为savedata23进入固定日志顺序，不是字节编号。  Port=23
      settings: AttributesFormatString=BeiYong2（保留记录项23）
  BeiYong3 : Outport  Description=记录项24 BeiYong3：备用常量0。作为savedata24进入固定日志顺序，不是字节编号。  Port=24
      settings: AttributesFormatString=BeiYong3（保留记录项24）
  BeiYong4 : Outport  Description=记录项25 BeiYong4：备用常量0。作为savedata25进入固定日志顺序，不是字节编号。  Port=25
      settings: AttributesFormatString=BeiYong4（保留记录项25）
  wires:
  S_SPM/1 -> [S_SPM]
  S_ClM_Parameter/1 -> Terminator/1
  S_MAlarm/1 -> [MAlarm]
  S_Servo_Out/1 -> [S_Servo_Out]
  [S_SPM] -> Bus Selector13/1
  Data Type Conversion19/1 -> ZhiLingHuiChuan/1
  Bus Selector13/1 -> Data Type Conversion19/1  "<Instr_XianShi（指令回显）>"
  [S_SPM] -> Bus Selector1/1
  Data Type Conversion1/1 -> T0/1
  Bus Selector1/1 -> Data Type Conversion1/1  "<T0（入口总温）>"
  Bus Selector3/1 -> Data Type Conversion2/1  "<Vpower（电源电压）>"
  [S_SPM] -> Bus Selector3/1
  Data Type Conversion2/1 -> dianyuandianya/1
  [S_SPM] -> Bus Selector2/1
  Bus Selector2/1 -> Data Type Conversion3/1  "<T4_Filter（滤波后排气温度）>"
  Bus Selector2/2 -> Data Type Conversion4/1  "<POil_Filter（滤波后燃油压力）>"
  Data Type Conversion3/1 -> T4/1
  Data Type Conversion4/1 -> POil/1
  S_EngineState/1 -> [EngineState]
  Product3/1 -> Data Type Conversion20/1
  Product7/1 -> Data Type Conversion22/1
  Bus Selector10/2 -> Product3/3  "<EValve_Cycle（主油阀周期计数）>"
  dth = T0-288.13/1 -> Product3/2
  Bus Selector10/1 -> Product3/1  "<EValve_Open（主油阀开通计数）>"
  Data Type Conversion20/1 -> EValve/1
  Data Type Conversion22/1 -> Eblast/1
  Bus Selector10/4 -> Product7/3  "<Eblast_Cycle（副油阀周期计数）>"
  dth = T0-288.9/1 -> Product7/2
  Bus Selector10/3 -> Product7/1  "<Eblast_Open（副油阀开通计数）>"
  [S_Servo_Out] -> Bus Selector10/1
  [S_SPM] -> Bus Selector17/1
  Bus Selector17/1 -> Data Type Conversion5/1  "<HuanSuanZhuanSu（温度修正转速）>"
  Data Type Conversion5/1 -> HuanSuanZhuanSu/1
  [S_SPM] -> Bus Selector14/1
  Bus Selector14/1 -> Logical Operator/1  "<SWI_Firework（点火器告警反馈）>"
  Bus Selector14/4 -> Logical Operator3/1  "<SWI_BleedAir（引气阀反馈）>"
  Bus Selector14/2 -> Logical Operator1/1  "<SWI_EValve（主油阀反馈）>"
  Bus Selector14/3 -> Logical Operator2/1  "<SWI_Eblast（副油阀反馈）>"
  Sum of Elements4/1 -> Data Type Conversion24/1
  Logical Operator/1 -> Gain2/1
  Logical Operator1/1 -> Gain3/1
  Logical Operator2/1 -> Gain4/1
  Logical Operator3/1 -> Gain5/1
  [S_Servo_Out] -> Bus Selector11/1
  Gain1/1 -> Sum of Elements4/1
  Gain6/1 -> Sum of Elements4/2
  Gain7/1 -> Sum of Elements4/3
  Gain8/1 -> Sum of Elements4/4
  Gain2/1 -> Sum of Elements4/5
  Gain3/1 -> Sum of Elements4/6
  Gain4/1 -> Sum of Elements4/7
  Gain5/1 -> Sum of Elements4/8
  Bus Selector11/1 -> Gain1/1  "<SWO_Firework（点火器使能）>"
  Bus Selector11/2 -> Gain6/1  "<EValve_Enable（主油阀使能）>"
  Bus Selector11/3 -> Gain7/1  "<Eblast_Enable（副油阀使能）>"
  Bus Selector11/4 -> Gain8/1  "<SWO_BleedAir（引气阀使能）>"
  Data Type Conversion24/1 -> KaiGuanLiang/1
  Bus Selector4/1 -> Data Type Conversion6/1  "<Origin_Nc（原位转速）>"
  Data Type Conversion6/1 -> WuLiZhuanSu/1
  [S_SPM] -> Bus Selector4/1
  [S_Servo_Out] -> Bus Selector15/1
  Bus Selector15/1 -> Data Type Conversion7/1  "<Accelerator（油泵给定控制量）>"
  Data Type Conversion7/1 -> NBump_MuBiao/1
  Product1/1 -> Data Type Conversion8/1
  dth = T0-288.1/1 -> Product1/2
  Bus Selector10/5 -> Product1/1  "<Motor_Open（起动电机开通计数）>"
  Bus Selector10/6 -> Product1/3  "<Motor_Cycle（起动电机周期计数）>"
  Data Type Conversion8/1 -> Motor/1
  [EngineState] -> Data Type Conversion9/1
  Data Type Conversion9/1 -> FaDongJiZhuangTai/1
  [MAlarm] -> Bus Selector9/1
  Sum of Elements1/1 -> Data Type Conversion16/1
  Gain9/1 -> Sum of Elements1/1
  Gain14/1 -> Sum of Elements1/2
  Gain15/1 -> Sum of Elements1/3
  Gain16/1 -> Sum of Elements1/4
  Gain10/1 -> Sum of Elements1/5
  Gain11/1 -> Sum of Elements1/6
  Gain12/1 -> Sum of Elements1/7
  Gain13/1 -> Sum of Elements1/8
  Bus Selector9/1 -> Gain9/1  "<Alarm_OverTemp（超温告警）>"
  Bus Selector9/2 -> Gain14/1  "<Alarm_OverSpeed（超转告警）>"
  Bus Selector9/3 -> Gain15/1  "<Flag_NcFailure（转速传感器故障标志）>"
  Bus Selector9/4 -> Gain16/1  "<Alarm_ECUReset（控制器复位告警）>"
  Bus Selector9/5 -> Gain10/1  "<Alarm_Vpower_Low（电源欠压告警）>"
  [S_SPM] -> Bus Selector18/1
  Bus Selector18/1 -> Gain11/1  "<SWI_ValveErr（阀门综合告警反馈）>"
  dth = T0-288.2/1 -> Gain12/1
  dth = T0-288.10/1 -> Gain13/1
  Data Type Conversion16/1 -> GuZhangXingXi/1
  [S_SPM] -> Bus Selector12/1
  Data Type Conversion11/1 -> Tecu/1
  Bus Selector12/1 -> Data Type Conversion11/1  "<Tecu（处理器温度）>"
  [S_SPM] -> Bus Selector8/1
  Data Type Conversion12/1 -> DianYuan/1
  Bus Selector8/1 -> Data Type Conversion12/1  "<SpeedLoad（装订转速）>"
  Bus Selector8/2 -> Data Type Conversion13/1  "<H_Gprs（导航高度）>"
  Bus Selector8/3 -> Data Type Conversion14/1  "<AirSpeed（飞行空速）>"
  Data Type Conversion13/1 -> H/1
  Data Type Conversion14/1 -> speed/1
  dth = T0-288.4/1 -> ZhuFaShuChu/1
  dth = T0-288.5/1 -> 12/1
  dth = T0-288.6/1 -> BeiYong1/1
  dth = T0-288.7/1 -> BeiYong2/1
  dth = T0-288.8/1 -> BeiYong3/1
  dth = T0-288.11/1 -> BeiYong4/1
  Data Type Conversion15/1 -> zhenjishu/1
  Hold/1(Out) -> Data Type Conversion15/1
